simulink model "course_lab3_example4"  (R2024b)
settings: Solver=ode45  StartTime=0.0  StopTime=5  MaxStep=0.003333333333333334  RelTol=1e-7  AbsTol=1e-9
model workspace (MAT data in the model file):
  A = 1
  K = 1
  den = [1 2 10]
  frequency = 1
  num = [0 0 10]
  web_input = timeseries
  web_input.Name = 'unnamed'
  web_input.DataInfo = tsdata.datametadata
  web_input.DataInfo.Interpolation = tsdata.interpolation
  web_input.DataInfo.Interpolation.Fhandle : function handle (value not decoded)
  web_input.DataInfo.Interpolation.Name = 'linear'
  web_input.TimeInfo = tsdata.timemetadata
  web_input.TimeInfo.Length = 1501
  web_input.TimeInfo.DuplicateTimes = 0
  web_input.TimeInfo.Time_ = [0 0.00333333333333 0.00666666666667 0.01 0.0133333333333 0.0166666666667 0.02 0.0233333333333 0.0266666666667 0.03 0.0333333333333 0.0366666666667 ... (1501 elements, 1501x1)]
  web_input.TimeInfo.Initialized = 1
  web_input.QualityInfo = tsdata.qualmetadata
  web_input.Data_ = [5 5.00675555556 5.01368888889 5.0208 5.02808888889 5.03555555556 5.0432 5.05102222222 5.05902222222 5.0672 5.07555555556 5.08408888889 ... (1501 elements, 1501x1)]
  wn = 10
  zeta = 0.5
settings Model: Creator=33657  LastModifiedBy=33657

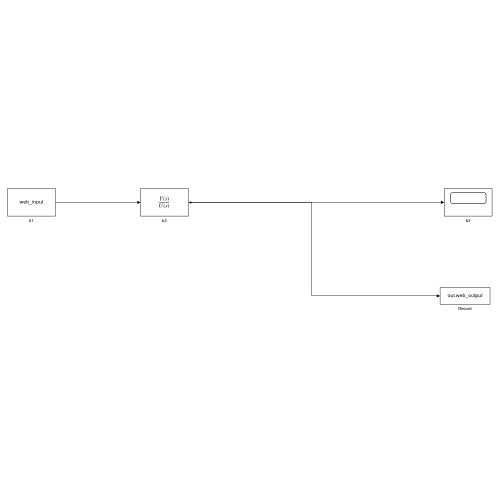
[thumbnail: Simulink's stored preview of the top-level diagram]
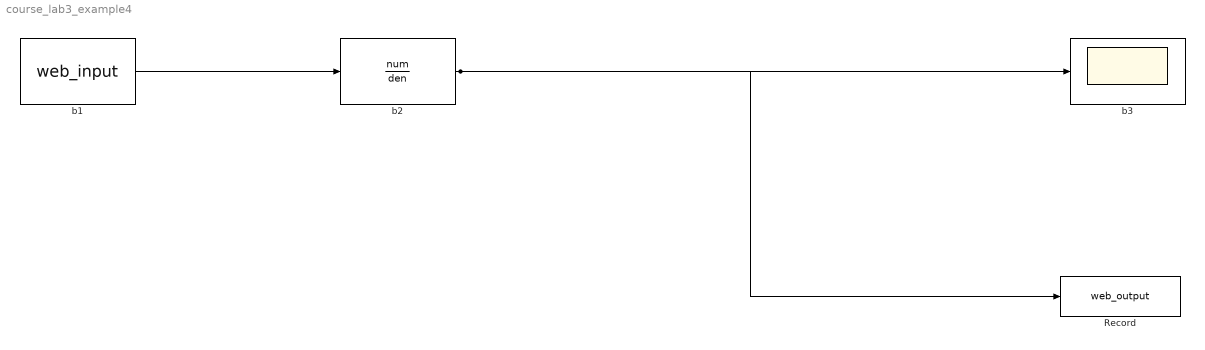
== system course_lab3_example4 ==
  Record : ToWorkspace  VariableName=web_output  SaveFormat=Timeseries  SampleTime=-1
  b1 : FromWorkspace  VariableName=web_input
  b2 : TransferFcn  Numerator=num  Denominator=den
  b3 : Scope
  wires:
  b1/1 -> b2/1
  b2/1 -> b3/1, Record/1
